simulink model "Control_LIM_H9"  (R2025b)
settings: Solver=VariableStepAuto  StartTime=0.0  StopTime=10  RelTol=1e-3
undefined symbols (not defined in the file): a, airgap, b, corriente, dent_lsm, force_lsm, frecuencia_acel, frecuencia_freno, fuerza, fuerza_drag, FuerzaX_freno, kd, magnitude, masa_pod, paso_polar, r, slip, vel_motor_freno, velocidad_drag
libraries: slpidlib x3, eeTransforms x1
(part 2 of 2)

== matlab function Control_LIM_H9/Modelado completo del motor DLIM/LIM Model/Equivalente eléctrico/Cálculo Máximo/MATLAB Function ==
  settings: updateMethod=DISCRETE
  data: frecuencia input; maximo output; valores input; tiempo input
function maximo = pico(frecuencia, valores, tiempo)

persistent antiguo_maximo
    if isempty(antiguo_maximo)
        antiguo_maximo = 0;
    end

persistent t_maximo
    if isempty(t_maximo)
        t_maximo = 0;
    end

persistent posible_nuevo_maximo
    if isempty(posible_nuevo_maximo)
        posible_nuevo_maximo = 0;
    end

persistent posible_t_maximo
    if isempty(posible_t_maximo)
        posible_t_maximo = 0;
    end


periodo = 1 / abs(frecuencia);
valor = max(abs(valores));


if valor >= antiguo_maximo
    maximo = valor;
    antiguo_maximo = valor;
    t_maximo = tiempo;
    posible_nuevo_maximo = 0;                           %Por qué?
    posible_t_maximo = tiempo;

else
    maximo = antiguo_maximo;

    if tiempo > t_maximo + 0.1 * periodo                        % Máxima diferencia de potencial en el periodo?
        if valor > posible_nuevo_maximo
            posible_nuevo_maximo = valor;
            posible_t_maximo = tiempo;
        end
    end

    if tiempo > t_maximo + 0.6 * periodo                        % Máxima diferencia de potencial en el periodo?
        maximo = posible_nuevo_maximo;                  % No habría que evaluar aquí también si el valor es mayor a posible_nuevo_maximo?
        antiguo_maximo = posible_nuevo_maximo;
        posible_nuevo_maximo = 0;
        t_maximo = posible_t_maximo;
    end
end

== matlab function Control_LIM_H9/Modelado completo del motor DLIM/LIM Model/Dinámica del Vehículo/MATLAB Function ==
  data: estado input; fuerza input double; fuerza_con_drag input; fuerza_total_real output double
function fuerza_total_real = fcn(estado, fuerza, fuerza_con_drag)

if estado == 7
    fuerza_total_real = fuerza;
else
    fuerza_total_real = fuerza_con_drag;
end

== matlab function Control_LIM_H9/Modelado completo del motor DLIM/LIM Model/Dinámica del Vehículo/MATLAB Function1 ==
  data: drag input; run input; drag_aero output
function drag_aero = fcn(drag, run)

if run == 3
    drag_aero = drag * 20;
else
    drag_aero = drag;
end

== matlab function Control_LIM_H9/Modelado completo del motor DLIM/LIM Model/Dinámica del Vehículo/MATLAB Function2 ==
  data: fuerza_x input double; fuerza_total output; fuerza_lsm input; run input; estado input
function fuerza_total = fcn(fuerza_x, fuerza_lsm, run, estado)

if run ~= 3 
   if estado == 1 && run == 2
       fuerza_total = fuerza_lsm;
   else
       fuerza_total = fuerza_x + fuerza_lsm;
   end

elseif estado == 6
    fuerza_total = fuerza_x;
else
    fuerza_total = fuerza_x;
end

== matlab function Control_LIM_H9/Modelado completo del motor DLIM/Cálculo Velocidad/MATLAB Function ==
  data: vel1 input; vel2 input; run input; vel output
function vel = fcn(vel1, vel2, run)

if run == 2
    vel = vel2;
else
    vel = vel1;
end

== matlab function Control_LIM_H9/Modelado completo del motor DLIM/Sensor IMU/MATLAB Function1 ==
  data: vel1 input; vel2 input; run input; vel output
function vel = fcn(vel1, vel2, run)

if run == 2
    vel = vel2;
else
    vel = vel1;
end

== matlab function Control_LIM_H9/Modelado completo del motor DLIM/LIM Model/Velocidad Real/MATLAB Function ==
  data: vel1 input; vel2 input; run input; vel output
function vel = fcn(vel1, vel2, run)

if run == 2
    vel = vel2;
else
    vel = vel1;
end

== matlab function Control_LIM_H9/Modelado completo del motor DLIM/LIM Model/Dinámica del Vehículo/MATLAB Function3 ==
  data: drag_in input; drag_out output; tiempo input
function drag_out = fcn(drag_in, tiempo)

if tiempo < 1
    drag_out = 0;
else
    drag_out = drag_in;
end



% Para que no se vaya hacia atrás antes de entrar en el booster

== matlab function Control_LIM_H9/Control de Velocidad/MATLAB Function1 ==
  data: abs input; i output; normal input; estado input
function i = fcn(abs, normal, estado)

if estado == 6
    i = abs;
else
    i = normal;
end

== matlab function Control_LIM_H9/Referencia Velocidad/MATLAB Function ==
  settings: updateMethod=DISCRETE
  data: pos input; tiempo input; vel input; estado output; corriente_pico input; metros_a_frenar input; vel_ref output; run input
function [estado, vel_ref] = fcn(pos, tiempo, vel, corriente_pico, metros_a_frenar, run)

persistent estado_sig
        if isempty(estado_sig) && run ~= 2
            estado_sig = 0;   
        elseif isempty(estado_sig)
            estado_sig = 1;
        end

 vel_ref = 0;
 estado = estado_sig;

%% Run 1: LIM + Booster

if run == 1

    vel_ref_deseada = 50;
        
    switch estado_sig
        case 0
            if tiempo > 1 && tiempo < 2
                estado_sig = 2;
                vel_ref = vel_ref_deseada;
            end
    
        case 2
            if pos > 6
                estado_sig = 4;
            end
            vel_ref = vel_ref_deseada;
    
    % Velocidad Crucero
        case 4
            if pos > 48 - metros_a_frenar  ||   vel > vel_ref_deseada        % En principio no debería hacer falta "vel > vel_ref_deseada" y el control debería mantenerse en crucero
                estado_sig = 7;
            end
            vel_ref = vel_ref_deseada;

    % Realmente frenado mecánico
        case 7                                                               % Estado inventado (como todos) que activa el frenado mecánico
            if vel < 1
                estado_sig = 0;
            end
            vel_ref = 0;
    end
end


%% Run 2: Booster

if run == 2

    vel_ref_deseada = 25;
        
    switch estado_sig
        
        case 0
            if tiempo > 1 && tiempo < 2
                estado_sig = 1;
                vel_ref = 0;
            end
        
        case 1
            if pos > 4.5
                estado_sig = 4;
            end
            vel_ref = vel_ref_deseada;
    

            % Velocidad Crucero
        case 4
            if pos > 48 - metros_a_frenar  ||   vel > 30
                estado_sig = 5;
            end
            vel_ref = vel_ref_deseada;

        case 5
            if vel <= 0
                estado_sig = 0;
            end
            vel_ref = 0;
    end
end


%% Run 3: Tubo

if run == 3

    vel_ref_deseada = 5;
        
    switch estado_sig
        case 0
            if tiempo > 1 && tiempo < 2
                estado_sig = 4;
                vel_ref = vel_ref_deseada;
            end

        % Velocidad Crucero
        case 4
            if pos > 7         % Frena 3 metros antes de los 10
                estado_sig = 6;
            end
            vel_ref = vel_ref_deseada;

        case 6
            if pos < 3
                estado_sig = 0;
            end
            vel_ref = -vel_ref_deseada;
    end
end

%% Run 4: LIM

if run == 4

    vel_ref_deseada = 35;
        
    switch estado_sig
        case 0
            if tiempo > 1 && tiempo < 2
                estado_sig = 2;
                vel_ref = vel_ref_deseada;
            end
    
        case 2
            if vel > vel_ref_deseada
                estado_sig = 4;
            end
            vel_ref = vel_ref_deseada;
    
    % Velocidad Crucero
        case 4
            if pos > 48 - metros_a_frenar  %||   vel > vel_ref_deseada
                estado_sig = 5;
            end
            vel_ref = vel_ref_deseada;

            case 5
            if vel <= 0
                estado_sig = 0;
            end
            vel_ref = 0;

    % Realmente frenado mecánico
        case 7                                                               % Estado inventado (como todos) que activa el frenado mecánico
            if vel < 1
                estado_sig = 0;
            end
            vel_ref = 0;
    end
end

== matlab function Control_LIM_H9/Control de Frecuencia/MATLAB Function ==
  data: vel input; frecuencia output; a input; b input
function frecuencia = fcn(vel, a, b)

frecuencia = a*vel + b;                       %ES una ecuación de la recta utilizando las constantes de la recta del ajuste de mínimos cuadrados de los picos de fuerza para cada frecuencia y velocidad.

== matlab function Control_LIM_H9/Control de Frecuencia/MATLAB Function1 ==
  data: f_acel input; f output; f_frenado input; estado input
function f = fcn(f_acel, f_frenado, estado)

if estado == 5 || estado == 0 || estado == 7            % la frecuencia no actúa con el estado 7
    f = f_frenado;
else
    f = f_acel;
end

== matlab function Control_LIM_H9/Modelado completo del motor DLIM/Sensor IMU/MATLAB Function ==
  data: valor input; valor_discretizado output; num_bits input; max input
function valor_discretizado = fcn(valor, num_bits, max)

min = -max;

if valor > max
    valor_discretizado = max;
    return
end

if valor < min
    valor_discretizado = min;
    return
end


num_valores = 2^num_bits;
valor_escalon = (max-min)/(num_valores-1);

i = min;

while (i < max)
    if (i + valor_escalon/2 > valor)
        valor_discretizado = i;
        return
    end
    i = i + valor_escalon;

end

valor_discretizado = max;

end

== matlab function Control_LIM_H9/Control de Corriente/MATLAB Function ==
  data: pico_voltaje output; corriente input; estado input; reset output
function [pico_voltaje, reset] = fcn(corriente, estado)

if estado == 0 || estado == 7 %|| estado == 5 
    pico_voltaje = 0;
    reset = 1;

else
    pico_voltaje = corriente;
    reset = 0;
end

== matlab function Control_LIM_H9/Modelado completo del motor DLIM/Cálculo Máximo/MATLAB Function ==
  settings: updateMethod=DISCRETE
  data: frecuencia input; maximo output; valores input; tiempo input
function maximo = pico(frecuencia, valores, tiempo)

persistent antiguo_maximo
    if isempty(antiguo_maximo)
        antiguo_maximo = 0;
    end

persistent t_maximo
    if isempty(t_maximo)
        t_maximo = 0;
    end

persistent posible_nuevo_maximo
    if isempty(posible_nuevo_maximo)
        posible_nuevo_maximo = 0;
    end

persistent posible_t_maximo
    if isempty(posible_t_maximo)
        posible_t_maximo = 0;
    end


periodo = 1 / abs(frecuencia);
valor = max(abs(valores));


if valor >= antiguo_maximo
    maximo = valor;
    antiguo_maximo = valor;
    t_maximo = tiempo;
    posible_nuevo_maximo = 0;
    posible_t_maximo = tiempo;

else
    maximo = antiguo_maximo;

    if tiempo > t_maximo + 0.1 * periodo
        if valor > posible_nuevo_maximo
            posible_nuevo_maximo = valor;
            posible_t_maximo = tiempo;
        end
    end

    if tiempo > t_maximo + 0.6 * periodo
        maximo = posible_nuevo_maximo;
        antiguo_maximo = posible_nuevo_maximo;
        posible_nuevo_maximo = 0;
        t_maximo = posible_t_maximo;
    end
end

== matlab function Control_LIM_H9/Modelado completo del motor DLIM/Sensor de Corriente/Sensor corriente U/Sensor ==
  data: I input; V output; Offset input
function V = fcn(I, Offset)

Vcc = 5;                                        %Vcc ??                             La corriente va hasta máximo 5V

if (I > 300)
    I = 300;
end

if (I < -300)
    I = -300;
end


V_ref = Vcc / 2;

V = V_ref + 0.005 * I;

V = V + Offset;                 % Por?


end

== matlab function Control_LIM_H9/Modelado completo del motor DLIM/Sensor de Corriente/Sensor corriente U/Discretizado Amplitud ==
  data: valor input; valor_discretizado output; num_valores input; max input; min input
function valor_discretizado = fcn(valor, num_valores, max, min)

if valor > max
    valor_discretizado = max;
    return
end

if valor < min
    valor_discretizado = min;
    return
end


valor_escalon = (max - min)/(num_valores - 1);


i = min;


while (i < max)
    if (i + valor_escalon/2 > valor)
        valor_discretizado = i;
        return
    end

    i = i + valor_escalon;
end


valor_discretizado = max;

end
